simulink model "Integrated_Transformer_SA1_fixed"  (R2025a)
settings: Solver=VariableStepAuto  StartTime=0.0  StopTime=86400  MaxStep=60  RelTol=1e-3
values from neighbouring files (symbols this model uses):
  B = 135.9/26.92    (= 5.04829123328)    [Case2_inputs.m]
  I_rated = S_rated/(sqrt(3)*V_rated)    [Case2_inputs.m]
  m = 0.8    [Case2_inputs.m]
  n = 0.8    [Case2_inputs.m]
  PEC_R = 0.42    [Case2_inputs.m]
  T_amb = 24    [Case2_inputs.m]    (also in run_SA1.m = T_list(i))
  Theta_H_0 = 24    [Case2_inputs.m]    (also in run_SA1.m = h(end); step12_ambient_vs_harmonics_datasheet.m = r{5}(end) + (Ta_const - 24))
  THETA_H_R = 18    [Case2_inputs.m]
  THETA_O_R = 49    [Case2_inputs.m]
  Theta_TO_0 = 24    [Case2_inputs.m]    (also in run_SA1.m = to(end); step12_ambient_vs_harmonics_datasheet.m = r{4}(end) + (Ta_const - 24))
  Tt_O = 180    [Case2_inputs.m]
  Tw_H = 6    [Case2_inputs.m]
undefined symbols (not defined in the file or in its folder): D1, Delta
libraries: spsThreePhaseParallelRLCLoadLib x5, spsThreePhaseBreakerLib x4, spsThreePhaseVIMeasurementLib x1, spsThreePhaseSourceLib x1, spsThreePhaseTransformerInductanceMatrixTypeTwoWindingsLib x1, spspowerguiLib x1
settings Model: Creator=Mahammad  LastModifiedBy=Mahammad

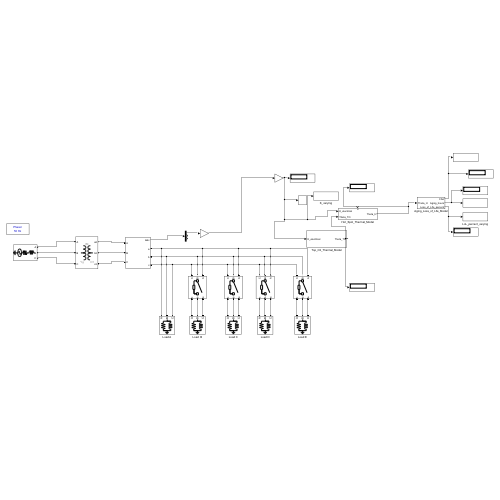
[thumbnail: Simulink's stored preview of the top-level diagram]
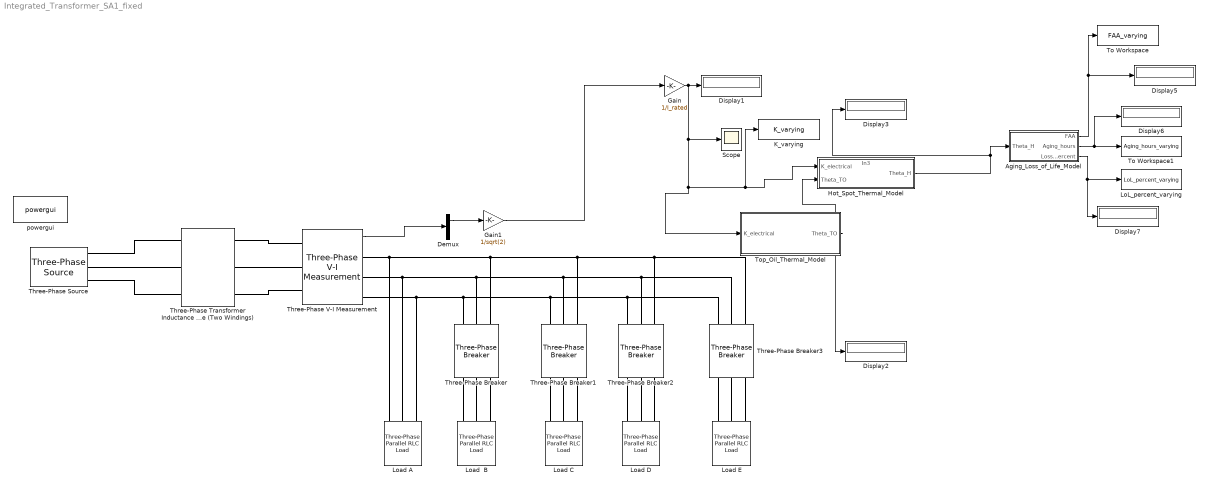
== system Integrated_Transformer_SA1_fixed ==
  Aging_Loss_of_Life_Model : Subsystem
  Demux : Demux  Outputs=3
  Display{1..3,5..7} (6 alike) : Display
  Gain : Gain  Gain=1/I_rated
  Gain1 : Gain  Gain=1/sqrt(2)
  Hot_Spot_Thermal_Model : Subsystem
      settings: PortSchema="{\"entries\":[{\"content\":{\"sides\":[{\"content\":{\"connectorIds\":[\"In1\",\"In2\"]},\"type\":\"ConnectorPlacement.EquallySpacedRectSide\",\"uuid\":\"0aa57ba8-0d68-4cb5-8658-c2847b7c0aff\"},{\"content\":{\"connectorIds\":[\"Out1\"],\"side\":\"RIGHT\"},\"type\":\"ConnectorPlacement.EquallySpacedRectSide\",\"uuid\":\"6e864665-ad43-47a8-b3b5-149113d94199\"},{\"content\":{\"connectorIds\":[\"In3\"],\"side\":\"TOP\"},\"type\":\"ConnectorPlacement.EquallySpacedRectSide\",\"uuid\":\"02735186-61f3-4675-b7d4-feeda3a9fdd1\"}]},\"type\":\"ConnectorPlacement.EquallySpacedConnector\",\"uuid\":\"40781f08-4b38-4a12-baa4-30e4b3f7e465\"}],\"packageUris\":[\"http://schema.mathworks.com/mf0/Connector/R2020b\"],\"version\":\"1.0\"}"
  K_varying : ToWorkspace  VariableName=K_varying  SaveFormat=Timeseries  SampleTime=-1
  LoL_percent_varying : ToWorkspace  VariableName=LoL_percent_varying  SaveFormat=Timeseries  SampleTime=-1
  Load  B : spsThreePhaseParallelRLCLoadLib/Three-Phase Parallel RLC Load  LConnTagsString=A|B|C  Configuration=Y (grounded)  NominalVoltage=10000  Vabc=[1e3 1e3 1e3]  Vabcp=[1e3 1e3 1e3]  NominalFrequency=50  UnbalancedPower=off  ActivePower=4.2795e6  InductivePower=2.0727e6  CapacitivePower=0  Pabc=[10e3 9e3 11e3]  QLabc=[100 90 110]  QCabc=[100 90 110]  Pabcp=[10e3 9e3 11e3]  QLabcp=[100 90 110]  QCabcp=[100 90 110]  Measurements=None  LoadType=constant Z
  Load A : spsThreePhaseParallelRLCLoadLib/Three-Phase Parallel RLC Load  LConnTagsString=A|B|C  Configuration=Y (grounded)  NominalVoltage=10000  Vabc=[1e3 1e3 1e3]  Vabcp=[1e3 1e3 1e3]  NominalFrequency=50  UnbalancedPower=off  ActivePower=32.4675e6  InductivePower=15.7247e6  CapacitivePower=0  Pabc=[10e3 9e3 11e3]  QLabc=[100 90 110]  QCabc=[100 90 110]  Pabcp=[10e3 9e3 11e3]  QLabcp=[100 90 110]  QCabcp=[100 90 110]  Measurements=None  LoadType=constant Z
  Load C : spsThreePhaseParallelRLCLoadLib/Three-Phase Parallel RLC Load  LConnTagsString=A|B|C  Configuration=Y (grounded)  NominalVoltage=10000  Vabc=[1e3 1e3 1e3]  Vabcp=[1e3 1e3 1e3]  NominalFrequency=50  UnbalancedPower=off  ActivePower=8.2890e6  InductivePower=4.0145e6  CapacitivePower=0  Pabc=[10e3 9e3 11e3]  QLabc=[100 90 110]  QCabc=[100 90 110]  Pabcp=[10e3 9e3 11e3]  QLabcp=[100 90 110]  QCabcp=[100 90 110]  Measurements=None  LoadType=constant Z
  Load D : spsThreePhaseParallelRLCLoadLib/Three-Phase Parallel RLC Load  LConnTagsString=A|B|C  Configuration=Y (grounded)  NominalVoltage=10000  Vabc=[1e3 1e3 1e3]  Vabcp=[1e3 1e3 1e3]  NominalFrequency=50  UnbalancedPower=off  ActivePower=7.9650e6  InductivePower=3.8576e6  CapacitivePower=0  Pabc=[10e3 9e3 11e3]  QLabc=[100 90 110]  QCabc=[100 90 110]  Pabcp=[10e3 9e3 11e3]  QLabcp=[100 90 110]  QCabcp=[100 90 110]  Measurements=None  LoadType=constant Z
  Load E : spsThreePhaseParallelRLCLoadLib/Three-Phase Parallel RLC Load  LConnTagsString=A|B|C  Configuration=Y (grounded)  NominalVoltage=10000  Vabc=[1e3 1e3 1e3]  Vabcp=[1e3 1e3 1e3]  NominalFrequency=50  UnbalancedPower=off  ActivePower=18.9990e6  InductivePower=9.2016e6  CapacitivePower=0  Pabc=[10e3 9e3 11e3]  QLabc=[100 90 110]  QCabc=[100 90 110]  Pabcp=[10e3 9e3 11e3]  QLabcp=[100 90 110]  QCabcp=[100 90 110]  Measurements=None  LoadType=constant Z
  Scope : Scope
      settings: ActiveDisplayYMinimum=0.69006519049080672  ActiveDisplayYMaximum=1.2108265583878102
  Three-Phase V-I Measurement : spsThreePhaseVIMeasurementLib/Three-Phase V-I Measurement  VoltageMeasurement=no  SetLabelV=off  LabelV=Vabc  Vpu=off  VpuLL=off  CurrentMeasurement=yes  SetLabelI=off  LabelI=Iabc  Ipu=off  Pbase=100e6  Vbase=500e3  OutputType=Magnitude  PhasorSimulation=on  PSBequivalent=0
  Three-Phase Breaker : spsThreePhaseBreakerLib/Three-Phase Breaker  InitialState=open  SwitchA=on  SwitchB=on  SwitchC=on  SwitchTimes=[21600]  External=off  BreakerResistance=0.01  SnubberResistance=1e6  SnubberCapacitance=inf  Measurements=None
  Three-Phase Breaker1 : spsThreePhaseBreakerLib/Three-Phase Breaker  InitialState=open  SwitchA=on  SwitchB=on  SwitchC=on  SwitchTimes=[43200 64800]  External=off  BreakerResistance=0.01  SnubberResistance=1e6  SnubberCapacitance=inf  Measurements=None
  Three-Phase Breaker2 : spsThreePhaseBreakerLib/Three-Phase Breaker  InitialState=open  SwitchA=on  SwitchB=on  SwitchC=on  SwitchTimes=[43200 64800]  External=off  BreakerResistance=0.01  SnubberResistance=1e6  SnubberCapacitance=inf  Measurements=None
  Three-Phase Breaker3 : spsThreePhaseBreakerLib/Three-Phase Breaker  InitialState=open  SwitchA=on  SwitchB=on  SwitchC=on  SwitchTimes=[90000]  External=off  BreakerResistance=0.01  SnubberResistance=1e6  SnubberCapacitance=inf  Measurements=None
  Three-Phase Source : spsThreePhaseSourceLib/Three-Phase Source  InternalConnection=Yg  VoltagePhases=off  Voltage=110e3  PhaseAngle=0  Voltage_phases=[25e3 25e3 25e3]/sqrt(3)  PhaseAngles_phases=[0 -120 +120]  Frequency=50  NonIdealSource=on  SpecifyImpedance=off  Resistance=0.8929  Inductance=16.58e-3  ShortCircuitLevel=100e6  BaseVoltage=110e3  XRratio=7  BusType=swing  Pref=10e3  Qref=0  Prefabc=[10e3, 10e3, 10e3]  Qrefabc=[0, 0, 0]  Qmin=-inf  Qmax=inf
  Three-Phase Transformer Inductance Matrix Type (Two Windings) : spsThreePhaseTransformerInductanceMatrixTypeTwoWindingsLib/Three-Phase Transformer Inductance Matrix Type (Two Windings)  CoreType=Three-limb or five-limb core  Winding1Connection=Yg  Winding2Connection=Delta (D1)  AutoTransformer=off  Measurements=None  NominalPower=[50e6, 50]  VLLnom=[110e3, 10.5e3]  WindingResistances=[0.01359, 0.01359]  NoLoadIexcPos=0.08424  NoLoadPlossPos=26920  ShortCircuitReactancePos=0.11207  ShortCircuitReactancePosAuto=0.06  NoLoadIexcZero=0.5  NoLoadPlossZero=1500  ShortCircuitReactanceZero=0.03  ShortCircuitReactanceZeroAuto=0.03
      settings: LibrarySourceBlock=|
      | sps_lib/Power Grid Elements/Three-Phase Transformer
      | Inductance Matrix Type
      | (Two Windings)
  To Workspace : ToWorkspace  VariableName=FAA_varying  SaveFormat=Timeseries  SampleTime=-1
  To Workspace1 : ToWorkspace  VariableName=Aging_hours_varying  SaveFormat=Timeseries  SampleTime=-1
  Top_Oil_Thermal_Model : Subsystem
  powergui : spspowerguiLib/powergui  Priority=1  SimulationMode=Phasor  SampleTime=50e-6  frequency=50  Iterations=50  frequencyindice=50  Pbase=100e6  ErrMax=1e-4  UnitsV=kV  UnitsW=MW  buscounter=0  FunctionMessages=off  echomessages=off  EnableUseOfTLC=off  CurrentSourceSwitches=off  DisableSnubberDevices=off  DisableRonSwitches=off  DisableVfSwitches=off  DisplayEquations=off  AutomaticDiscreteSolvers=off  SolverType=Tustin/Backward Euler (TBE)  Interpol=off  ExternalGateDelay=off  methode=off  Ts=100  x0status=blocks  SPID=on  SwTol=0  HookPort=off  NonlinearTolerance=1e-4  nMaxIteration=100  ContinueOnMaxIteration=off  RestoreLinks=warning  ResistiveCurrentMeasurement=off  Frange=[0:2:500]  Ylog=off  Xlog=on  ShowGrid=off  save=off  variable=ZData  structure=0  ZoomFFT=off  StartTime=0.0  cycles=1  DisplayStyle=1  fundamental=60  FreqAxis=off  MaxFrequency=1000  frequencyindicesteady=1  RmsSteady=1  display=off
  wires:
  Three-Phase V-I Measurement/1 -> Demux/1
  Demux/1 -> Gain1/1
  Gain/1 -> Scope/1, Top_Oil_Thermal_Model/1(K_electrical), K_varying/1, Hot_Spot_Thermal_Model/1(K_electrical), Display1/1
  Top_Oil_Thermal_Model/1(Theta_TO) -> Hot_Spot_Thermal_Model/2(Theta_TO), Display2/1
  Gain1/1 -> Gain/1
  Aging_Loss_of_Life_Model/1(FAA) -> To Workspace/1, Display5/1
  Aging_Loss_of_Life_Model/3(Loss_of_Life_percent) -> LoL_percent_varying/1, Display7/1
  Aging_Loss_of_Life_Model/2(Aging_hours) -> To Workspace1/1, Display6/1
  Hot_Spot_Thermal_Model/1(Theta_H) -> Display3/1, Aging_Loss_of_Life_Model/1(Theta_H)
  connections:
  Three-Phase Source/RConn1 -- Three-Phase Transformer Inductance Matrix Type (Two Windings)/LConn1
  Three-Phase Source/RConn2 -- Three-Phase Transformer Inductance Matrix Type (Two Windings)/LConn2
  Three-Phase Source/RConn3 -- Three-Phase Transformer Inductance Matrix Type (Two Windings)/LConn3
  Three-Phase Transformer Inductance Matrix Type (Two Windings)/RConn1 -- Three-Phase V-I Measurement/LConn1
  Three-Phase Transformer Inductance Matrix Type (Two Windings)/RConn2 -- Three-Phase V-I Measurement/LConn2
  Three-Phase V-I Measurement/LConn3 -- Three-Phase Transformer Inductance Matrix Type (Two Windings)/RConn3
  Load A/LConn1 -- Three-Phase Breaker3/LConn1 -- Three-Phase Breaker2/LConn1 -- Three-Phase Breaker1/LConn1 -- Three-Phase Breaker/LConn1 -- Three-Phase V-I Measurement/RConn1
  Load A/LConn2 -- Three-Phase Breaker3/LConn2 -- Three-Phase Breaker2/LConn2 -- Three-Phase Breaker1/LConn2 -- Three-Phase Breaker/LConn2 -- Three-Phase V-I Measurement/RConn2
  Load A/LConn3 -- Three-Phase Breaker3/LConn3 -- Three-Phase Breaker2/LConn3 -- Three-Phase Breaker1/LConn3 -- Three-Phase Breaker/LConn3 -- Three-Phase V-I Measurement/RConn3
  Three-Phase Breaker/RConn3 -- Load  B/LConn1
  Load  B/LConn2 -- Three-Phase Breaker/RConn2
  Three-Phase Breaker/RConn1 -- Load  B/LConn3
  Load C/LConn3 -- Three-Phase Breaker1/RConn1
  Load C/LConn1 -- Three-Phase Breaker1/RConn3
  Three-Phase Breaker1/RConn2 -- Load C/LConn2
  Load D/LConn3 -- Three-Phase Breaker2/RConn1
  Three-Phase Breaker2/RConn2 -- Load D/LConn2
  Load D/LConn1 -- Three-Phase Breaker2/RConn3
  Load E/LConn1 -- Three-Phase Breaker3/RConn3
  Three-Phase Breaker3/RConn2 -- Load E/LConn2
  Load E/LConn3 -- Three-Phase Breaker3/RConn1

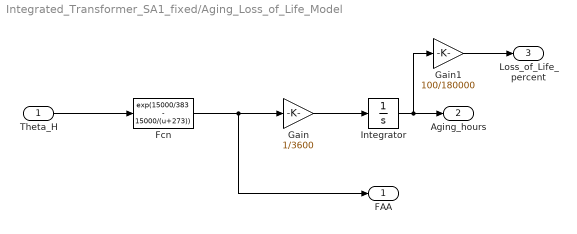
== system Integrated_Transformer_SA1_fixed/Aging_Loss_of_Life_Model ==
  Theta_H : Inport
  Fcn : Fcn  Expr=exp(15000/383 - 15000/(u+273))
  Gain : Gain  Gain=1/3600
  Gain1 : Gain  Gain=100/180000
  Integrator : Integrator
  FAA : Outport
  Aging_hours : Outport  Port=2
  Loss_of_Life_percent : Outport  Port=3
  wires:
  Theta_H/1 -> Fcn/1
  Fcn/1 -> Gain/1, FAA/1
  Gain/1 -> Integrator/1
  Integrator/1 -> Gain1/1, Aging_hours/1
  Gain1/1 -> Loss_of_Life_percent/1

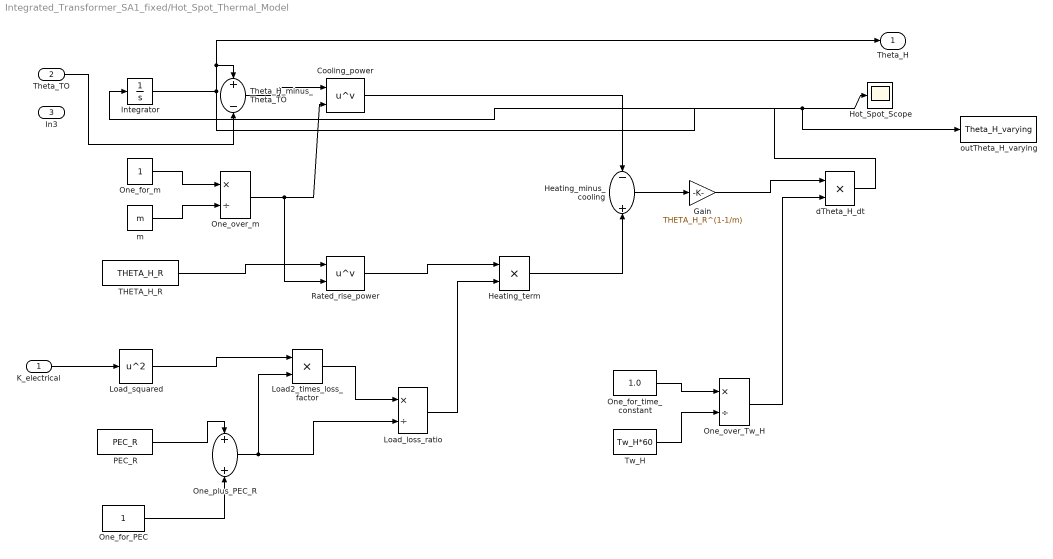
== system Integrated_Transformer_SA1_fixed/Hot_Spot_Thermal_Model ==
  K_electrical : Inport
  Theta_TO : Inport  Port=2
  In3 : Inport  Port=3
  Cooling_power : Math  Operator=pow  SignedPower=on
  Gain : Gain  Gain=THETA_H_R^(1-1/m)
  Heating_minus_cooling : Sum  Inputs=-+
  Heating_term : Product  Inputs=**
  Hot_Spot_Scope : Scope
      settings: ActiveDisplayYMinimum=-1  ActiveDisplayYMaximum=1
  Integrator : Integrator  InitialCondition=Theta_H_0
  Load2_times_loss_factor : Product  Inputs=**
  Load_loss_ratio : Product  Inputs=*/
  Load_squared : Math  Operator=square
  One_for_PEC : Constant
  One_for_m : Constant
  One_for_time_constant : Constant  Value=1.0
  One_over_Tw_H : Product  Inputs=*/
  One_over_m : Product  Inputs=*/
  One_plus_PEC_R : Sum
  PEC_R : Constant  Value=PEC_R
  Rated_rise_power : Math  Operator=pow  SignedPower=on
  THETA_H_R : Constant  Value=THETA_H_R
  Theta_H_minus_Theta_TO : Sum  Inputs=+-
  Tw_H : Constant  Value=Tw_H*60
  dTheta_H_dt : Product  Inputs=**
  m : Constant  Value=m
  outTheta_H_varying : ToWorkspace  VariableName=Theta_H_varying  SaveFormat=Structure With Time  SampleTime=-1
  Theta_H : Outport
  wires:
  Rated_rise_power/1 -> Heating_term/1
  Cooling_power/1 -> Heating_minus_cooling/1
  dTheta_H_dt/1 -> Integrator/1
  Theta_TO/1 -> Theta_H_minus_Theta_TO/2
  Theta_H_minus_Theta_TO/1 -> Cooling_power/1
  One_plus_PEC_R/1 -> Load2_times_loss_factor/2, Load_loss_ratio/2
  K_electrical/1 -> Load_squared/1
  One_over_m/1 -> Cooling_power/2, Rated_rise_power/2
  Integrator/1 -> Theta_H/1, Theta_H_minus_Theta_TO/1, outTheta_H_varying/1, Hot_Spot_Scope/1
  m/1 -> One_over_m/2
  Heating_term/1 -> Heating_minus_cooling/2
  Load2_times_loss_factor/1 -> Load_loss_ratio/1
  Tw_H/1 -> One_over_Tw_H/2
  One_for_m/1 -> One_over_m/1
  One_over_Tw_H/1 -> dTheta_H_dt/2
  PEC_R/1 -> One_plus_PEC_R/1
  Load_squared/1 -> Load2_times_loss_factor/1
  One_for_PEC/1 -> One_plus_PEC_R/2
  One_for_time_constant/1 -> One_over_Tw_H/1
  THETA_H_R/1 -> Rated_rise_power/1
  Load_loss_ratio/1 -> Heating_term/2
  Heating_minus_cooling/1 -> Gain/1
  Gain/1 -> dTheta_H_dt/1

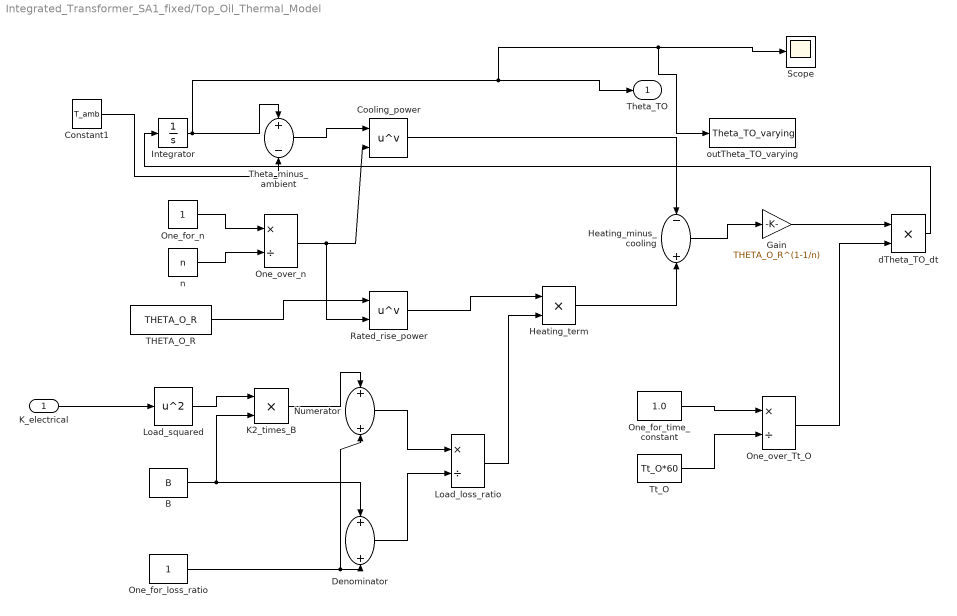
== system Integrated_Transformer_SA1_fixed/Top_Oil_Thermal_Model ==
  K_electrical : Inport
  B : Constant  Value=B
  Constant1 : Constant  Value=T_amb
  Cooling_power : Math  Operator=pow  SignedPower=on
  Denominator : Sum
  Gain : Gain  Gain=THETA_O_R^(1-1/n)
  Heating_minus_cooling : Sum  Inputs=-+
  Heating_term : Product  Inputs=**
  Integrator : Integrator  InitialCondition=Theta_TO_0
  K2_times_B : Product  Inputs=**
  Load_loss_ratio : Product  Inputs=*/
  Load_squared : Math  Operator=square
  Numerator : Sum
  One_for_loss_ratio : Constant
  One_for_n : Constant
  One_for_time_constant : Constant  Value=1.0
  One_over_Tt_O : Product  Inputs=*/
  One_over_n : Product  Inputs=*/
  Rated_rise_power : Math  Operator=pow  SignedPower=on
  Scope : Scope
      settings: ActiveDisplayYMinimum=-1  ActiveDisplayYMaximum=1
  THETA_O_R : Constant  Value=THETA_O_R
  Theta_minus_ambient : Sum  Inputs=+-
  Tt_O : Constant  Value=Tt_O*60
  dTheta_TO_dt : Product  Inputs=**
  n : Constant  Value=n
  outTheta_TO_varying : ToWorkspace  VariableName=Theta_TO_varying  SaveFormat=Structure With Time  SampleTime=-1
  Theta_TO : Outport
  wires:
  Integrator/1 -> Theta_TO/1, outTheta_TO_varying/1, Scope/1, Theta_minus_ambient/1
  dTheta_TO_dt/1 -> Integrator/1
  B/1 -> K2_times_B/2, Denominator/1
  Constant1/1 -> Theta_minus_ambient/2
  Cooling_power/1 -> Heating_minus_cooling/1
  One_over_n/1 -> Cooling_power/2, Rated_rise_power/2
  Load_squared/1 -> K2_times_B/1
  Tt_O/1 -> One_over_Tt_O/2
  Denominator/1 -> Load_loss_ratio/2
  One_for_time_constant/1 -> One_over_Tt_O/1
  Heating_term/1 -> Heating_minus_cooling/2
  One_for_loss_ratio/1 -> Numerator/2, Denominator/2
  K2_times_B/1 -> Numerator/1
  Theta_minus_ambient/1 -> Cooling_power/1
  Load_loss_ratio/1 -> Heating_term/2
  Rated_rise_power/1 -> Heating_term/1
  Numerator/1 -> Load_loss_ratio/1
  THETA_O_R/1 -> Rated_rise_power/1
  One_for_n/1 -> One_over_n/1
  n/1 -> One_over_n/2
  K_electrical/1 -> Load_squared/1
  One_over_Tt_O/1 -> dTheta_TO_dt/2
  Heating_minus_cooling/1 -> Gain/1
  Gain/1 -> dTheta_TO_dt/1
